simulink model "Power_Sensors"  (R2026b)
settings: Solver=VariableStepAuto
undefined symbols (not defined in the file or in its folder): DiscIntNeverNeededParam, P, Ts
libraries: eeGeneralControl x3, simulink x1
settings Model: Creator=aomar  LastModifiedBy=aomar

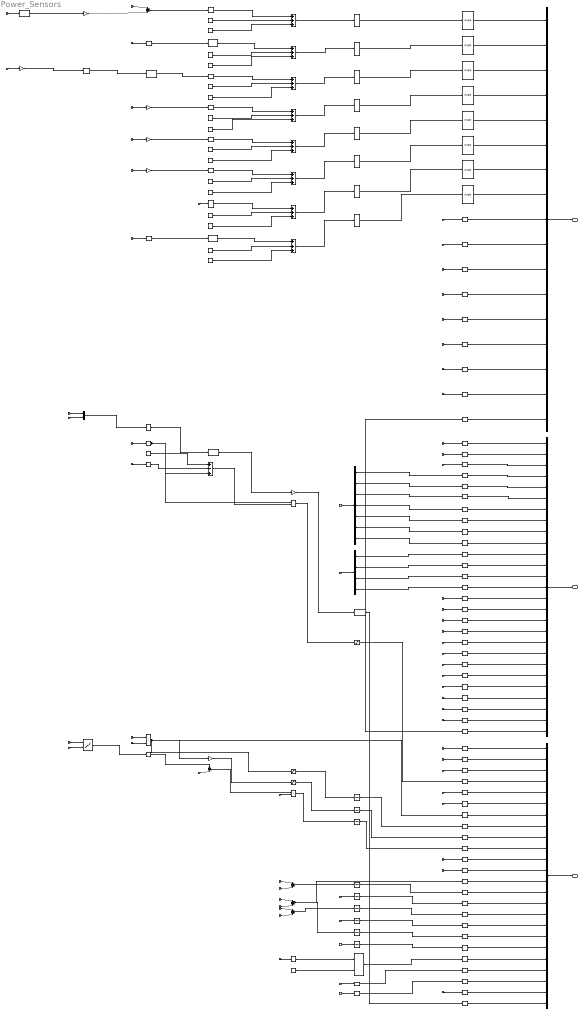
== system Power_Sensors ==
  pack_V_cell_true : Inport  PortName=pack  Element=V_cell_true
  pack_V_cell_true_2 : Inport  PortName=pack  Element=V_cell_true
  pack_T_cell_true : Inport  PortName=pack  Element=T_cell_true
  pack_T_cell_true_{2..5} (4 alike) : Inport  PortName=pack  Element=T_cell_true
  pack_SOC_true : Inport  PortName=pack  Element=SOC_true
  pack_SOC_true_2 : Inport  PortName=pack  Element=SOC_true
  pack_SOC_true_3 : Inport  PortName=pack  Element=SOC_true
  pack_SOC_true_4 : Inport  PortName=pack  Element=SOC_true
  thermal_T_air : Inport  Port=2  PortName=thermal  Element=T_air
  pdu_I_pack : Inport  Port=3  PortName=pdu  Element=I_pack
  pdu_I_pack_{2..6} (5 alike) : Inport  Port=3  PortName=pdu  Element=I_pack
  pdu_V_pack : Inport  Port=3  PortName=pdu  Element=V_pack
  pdu_V_pack_{2..5} (4 alike) : Inport  Port=3  PortName=pdu  Element=V_pack
  pdu_V_bus : Inport  Port=3  PortName=pdu  Element=V_bus
  pdu_V_bus_2 : Inport  Port=3  PortName=pdu  Element=V_bus
  pdu_V_dock : Inport  Port=3  PortName=pdu  Element=V_dock
  pdu_fuse_ok : Inport  Port=3  PortName=pdu  Element=fuse_ok
  pdu_K1_closed : Inport  Port=3  PortName=pdu  Element=K1_closed
  pdu_K1_closed_2 : Inport  Port=3  PortName=pdu  Element=K1_closed
  pdu_K1_closed_3 : Inport  Port=3  PortName=pdu  Element=K1_closed
  pdu_K2_closed : Inport  Port=3  PortName=pdu  Element=K2_closed
  pdu_K2_closed_2 : Inport  Port=3  PortName=pdu  Element=K2_closed
  pdu_K4_closed : Inport  Port=3  PortName=pdu  Element=K4_closed
  pdu_K4_closed_2 : Inport  Port=3  PortName=pdu  Element=K4_closed
  pdu_F_MAIN_ok : Inport  Port=3  PortName=pdu  Element=F_MAIN_ok
  pdu_P_trac_L : Inport  Port=3  PortName=pdu  Element=P_trac_L
  pdu_P_trac_R : Inport  Port=3  PortName=pdu  Element=P_trac_R
  pdu_P_bms : Inport  Port=3  PortName=pdu  Element=P_bms
  pdu_P_pdu_loss : Inport  Port=3  PortName=pdu  Element=P_pdu_loss
  pdu_P_chg_bus : Inport  Port=3  PortName=pdu  Element=P_chg_bus
  lv_fuse24_ok : Inport  Port=4  PortName=lv  Element=fuse24_ok
  lv_rails : Inport  Port=4  PortName=lv  Element=rails
  lv_rail_ok : Inport  Port=4  PortName=lv  Element=rail_ok
  lv_K3_closed : Inport  Port=4  PortName=lv  Element=K3_closed
  lv_P_lv : Inport  Port=4  PortName=lv  Element=P_lv
  lv_P_k3_loss : Inport  Port=4  PortName=lv  Element=P_k3_loss
  lv_P_dcdc_loss : Inport  Port=4  PortName=lv  Element=P_dcdc_loss
  lv_P_dcdc_loss_2 : Inport  Port=4  PortName=lv  Element=P_dcdc_loss
  safety_dock_present : Inport  Port=5  PortName=safety  Element=dock_present
  safety_dock_present_2 : Inport  Port=5  PortName=safety  Element=dock_present
  safety_Safety_OK : Inport  Port=5  PortName=safety  Element=Safety_OK
  safety_Safety_OK_2 : Inport  Port=5  PortName=safety  Element=Safety_OK
  safety_Safety_HV_OK : Inport  Port=5  PortName=safety  Element=Safety_HV_OK
  safety_Safety_HV_OK_2 : Inport  Port=5  PortName=safety  Element=Safety_HV_OK
  safety_key_on : Inport  Port=5  PortName=safety  Element=key_on
  safety_key_on_2 : Inport  Port=5  PortName=safety  Element=key_on
  safety_EStop_Any : Inport  Port=5  PortName=safety  Element=EStop_Any
  safety_EStop_Ch1_OK : Inport  Port=5  PortName=safety  Element=EStop_Ch1_OK
  safety_EStop_Ch2_OK : Inport  Port=5  PortName=safety  Element=EStop_Ch2_OK
  safety_Safety_Latched_Off : Inport  Port=5  PortName=safety  Element=Safety_Latched_Off
  impl_P_impl : Inport  Port=6  PortName=impl  Element=P_impl
  charger_P_grid : Inport  Port=7  PortName=charger  Element=P_grid
  env_T_amb : Inport  Port=8  PortName=env  Element=T_amb
  flt_bms_fault : Inport  Port=9  PortName=flt  Element=bms_fault
  BMS_Meas_BC : BusCreator  Inputs=17  OutDataTypeStr=Bus: Bus_BMS_Meas  NonVirtualBus=on
      settings: InheritFromInputs=off
  Fuse_Blown_u8 : DataTypeConversion  OutDataTypeStr=uint8  RndMeth=Nearest
  Fuse_ok : Mux  Inputs=2
  I_abs : Abs  SaturateOnIntegerOverflow=off
  I_peak : simulink/Math Operations/MinMax Running Resettable  Function=max  vinit=0.0
  I_peak_reset : Constant  Value=false  OutDataTypeStr=boolean  SampleTime=Ts.base
  Int_E_chg_bus : DiscreteIntegrator  gainval=1/3600  SampleTime=Ts.base  ICPrevOutput=DiscIntNeverNeededParam  ICPrevScaledInput=DiscIntNeverNeededParam
  Int_E_dcdc_loss : DiscreteIntegrator  gainval=1/3600  SampleTime=Ts.base  ICPrevOutput=DiscIntNeverNeededParam  ICPrevScaledInput=DiscIntNeverNeededParam
  Int_E_impl_dc : DiscreteIntegrator  gainval=1/3600  SampleTime=Ts.base  ICPrevOutput=DiscIntNeverNeededParam  ICPrevScaledInput=DiscIntNeverNeededParam
  Int_E_in : DiscreteIntegrator  gainval=1/3600  SampleTime=Ts.base  ICPrevOutput=DiscIntNeverNeededParam  ICPrevScaledInput=DiscIntNeverNeededParam
  Int_E_loss_batt : DiscreteIntegrator  gainval=1/3600  SampleTime=Ts.base  ICPrevOutput=DiscIntNeverNeededParam  ICPrevScaledInput=DiscIntNeverNeededParam
  Int_E_lv : DiscreteIntegrator  gainval=1/3600  SampleTime=Ts.base  ICPrevOutput=DiscIntNeverNeededParam  ICPrevScaledInput=DiscIntNeverNeededParam
  Int_E_out : DiscreteIntegrator  gainval=1/3600  SampleTime=Ts.base  ICPrevOutput=DiscIntNeverNeededParam  ICPrevScaledInput=DiscIntNeverNeededParam
  Int_E_pdu_loss : DiscreteIntegrator  gainval=1/3600  SampleTime=Ts.base  ICPrevOutput=DiscIntNeverNeededParam  ICPrevScaledInput=DiscIntNeverNeededParam
  Int_E_trac_dc : DiscreteIntegrator  gainval=1/3600  SampleTime=Ts.base  ICPrevOutput=DiscIntNeverNeededParam  ICPrevScaledInput=DiscIntNeverNeededParam
  Ipack_LPF : eeGeneralControl/Low-Pass Filter (Discrete or Continuous)  K=1  T=P.power.sensors.Ipack.tau  B=inf  A=-inf  init_option=Inherited from block input  x0=0  Ts=Ts.base
  Ipack_ZOH : ZeroOrderHold  SampleTime=Ts.afe
  Ipack_bias : Bias  Bias=P.power.sensors.Ipack.offset  SaturateOnIntegerOverflow=off
  Ipack_gain : Gain  Gain=1 + P.power.sensors.Ipack.gain_err
  Ipack_noise : RandomNumber  Mean=zeros(1,1)  Variance=P.power.sensors.Ipack.sigma^2  Seed=P.power.sensors.seed + 33  SampleTime=Ts.afe
  Ipack_offset : Constant  Value=0  SampleTime=Ts.afe
  Ipack_q : DataTypeConversion  OutDataTypeStr=single  SaturateOnIntegerOverflow=off  RndMeth=Floor
  Ipack_quant : Quantizer  QuantizationInterval=P.power.sensors.Ipack.q
  Ipack_sum : Sum  Inputs=+++
  OCV_lookup : Lookup_n-D  BreakpointsForDimension1=P.power.cell.SOC_bp  BreakpointsForDimension2=P.power.cell.T_bp  Table=P.power.cell.OCV_tab  ExtrapMethod=Clip  InternalRulePriority=Speed  RndMeth=Simplest
      settings: InputPortMap=u0,u1
  OCV_sum : Sum  Inputs=+
  P_in_pos : Saturate  UpperLimit=inf  LowerLimit=0
  P_loss_batt : Product
  P_lv_total : Sum
  P_neg : Gain  Gain=-1
  P_out_pos : Saturate  UpperLimit=inf  LowerLimit=0
  P_pack : Product
  P_pdu_total : Sum
  P_trac : Sum
  PowerStatus_BC : BusCreator  Inputs=27  OutDataTypeStr=Bus: Bus_PowerStatus  NonVirtualBus=on
      settings: InheritFromInputs=off
  PowerTruth_BC : BusCreator  Inputs=24  OutDataTypeStr=Bus: Bus_PowerTruth  NonVirtualBus=on
      settings: InheritFromInputs=off
  SOC_den : Sum  Inputs=+-+
  SOC_max : MinMax  Function=max
  SOC_min : MinMax
  SOC_pack_div : Product  Inputs=*/
  SOC_pack_sat : Saturate  UpperLimit=1  LowerLimit=0
  T_max : MinMax  Function=max
  T_min : MinMax
  Tair_NTC_lag : eeGeneralControl/Low-Pass Filter (Discrete or Continuous)  K=1  T=P.power.sensors.Tcell.tau  B=inf  A=-inf  init_option=Inherited from block input  x0=0  Ts=Ts.afe
  Tair_ZOH : ZeroOrderHold  SampleTime=Ts.afe
  Tair_noise : RandomNumber  Mean=zeros(1,1)  Variance=P.power.sensors.Tcell.sigma^2  Seed=P.power.sensors.seed + 37  SampleTime=Ts.afe
  Tair_offset : Constant  Value=0  SampleTime=Ts.afe
  Tair_q : DataTypeConversion  OutDataTypeStr=single  SaturateOnIntegerOverflow=off  RndMeth=Floor
  Tair_quant : Quantizer  QuantizationInterval=P.power.sensors.Tcell.q
  Tair_sum : Sum  Inputs=+++
  Tamb_RT : RateTransition  OutPortSampleTime=Ts.afe
  Tamb_noise : RandomNumber  Mean=zeros(1,1)  Variance=P.power.sensors.Tcell.sigma^2  Seed=P.power.sensors.seed + 38  SampleTime=Ts.afe
  Tamb_offset : Constant  Value=0  SampleTime=Ts.afe
  Tamb_q : DataTypeConversion  OutDataTypeStr=single  SaturateOnIntegerOverflow=off  RndMeth=Floor
  Tamb_quant : Quantizer  QuantizationInterval=P.power.sensors.Tcell.q
  Tamb_sum : Sum  Inputs=+++
  Tcell_NTC_lag : eeGeneralControl/Low-Pass Filter (Discrete or Continuous)  K=1  T=P.power.sensors.Tcell.tau  B=inf  A=-inf  init_option=Inherited from block input  x0=0  Ts=Ts.afe
  Tcell_ZOH : ZeroOrderHold  SampleTime=Ts.afe
  Tcell_noise : RandomNumber  Mean=zeros(P.power.pack.Ns,1)  Variance=P.power.sensors.Tcell.sigma^2  Seed=P.power.sensors.seed + (P.power.pack.Ns+1:2*P.power.pack.Ns)'  SampleTime=Ts.afe
  Tcell_offset : Constant  Value=P.power.sensors.Tcell.offset(:)  SampleTime=Ts.afe
  Tcell_q : DataTypeConversion  OutDataTypeStr=single  SaturateOnIntegerOverflow=off  RndMeth=Floor
  Tcell_quant : Quantizer  QuantizationInterval=P.power.sensors.Tcell.q
  Tcell_sum : Sum  Inputs=+++
  Vbus_ZOH : ZeroOrderHold  SampleTime=Ts.afe
  Vbus_gain : Gain  Gain=1 + P.power.sensors.Vpack.gain_err
  Vbus_noise : RandomNumber  Mean=zeros(1,1)  Variance=P.power.sensors.Vpack.sigma^2  Seed=P.power.sensors.seed + 35  SampleTime=Ts.afe
  Vbus_offset : Constant  Value=0  SampleTime=Ts.afe
  Vbus_q : DataTypeConversion  OutDataTypeStr=single  SaturateOnIntegerOverflow=off  RndMeth=Floor
  Vbus_quant : Quantizer  QuantizationInterval=P.power.sensors.Vpack.q
  Vbus_sum : Sum  Inputs=+++
  Vcell_ZOH : ZeroOrderHold  SampleTime=Ts.afe
  Vcell_fault : Sum
  Vcell_noise : RandomNumber  Mean=zeros(P.power.pack.Ns,1)  Variance=P.power.sensors.Vcell.sigma^2  Seed=P.power.sensors.seed + (1:P.power.pack.Ns)'  SampleTime=Ts.afe
  Vcell_offset : Constant  Value=P.power.sensors.Vcell.offset(:)  SampleTime=Ts.afe
  Vcell_q : DataTypeConversion  OutDataTypeStr=single  SaturateOnIntegerOverflow=off  RndMeth=Floor
  Vcell_quant : Quantizer  QuantizationInterval=P.power.sensors.Vcell.q
  Vcell_sum : Sum  Inputs=+++
  Vdock_ZOH : ZeroOrderHold  SampleTime=Ts.afe
  Vdock_gain : Gain  Gain=1 + P.power.sensors.Vpack.gain_err
  Vdock_noise : RandomNumber  Mean=zeros(1,1)  Variance=P.power.sensors.Vpack.sigma^2  Seed=P.power.sensors.seed + 36  SampleTime=Ts.afe
  Vdock_offset : Constant  Value=0  SampleTime=Ts.afe
  Vdock_q : DataTypeConversion  OutDataTypeStr=single  SaturateOnIntegerOverflow=off  RndMeth=Floor
  Vdock_quant : Quantizer  QuantizationInterval=P.power.sensors.Vpack.q
  Vdock_sum : Sum  Inputs=+++
  Vpack_ZOH : ZeroOrderHold  SampleTime=Ts.afe
  Vpack_gain : Gain  Gain=1 + P.power.sensors.Vpack.gain_err
  Vpack_noise : RandomNumber  Mean=zeros(1,1)  Variance=P.power.sensors.Vpack.sigma^2  Seed=P.power.sensors.seed + 34  SampleTime=Ts.afe
  Vpack_offset : Constant  Value=0  SampleTime=Ts.afe
  Vpack_q : DataTypeConversion  OutDataTypeStr=single  SaturateOnIntegerOverflow=off  RndMeth=Floor
  Vpack_quant : Quantizer  QuantizationInterval=P.power.sensors.Vpack.q
  Vpack_sum : Sum  Inputs=+++
  bms_fault_V : Gain  Gain=[0.5; zeros(P.power.pack.Ns-1,1)]
  bms_fault_dbl : DataTypeConversion  OutDataTypeStr=double  SaturateOnIntegerOverflow=off  RndMeth=Floor
  dV_internal : Sum  Inputs=+-
  fuse_bits_dbl : DataTypeConversion  OutDataTypeStr=double  SaturateOnIntegerOverflow=off  RndMeth=Floor
  fuse_blown_bits : Logic  Operator=NOT  AllPortsSameDT=off  OutDataTypeStr=boolean
  fuse_weights : Gain  Gain=2.^(0:6)  Multiplication=Matrix(K*u)
  meas_Dock_Present : ZeroOrderHold  SampleTime=Ts.afe
  meas_FuseMain_OK : ZeroOrderHold  SampleTime=Ts.afe
  meas_Fuse_Blown : ZeroOrderHold  SampleTime=Ts.afe
  meas_K1_fb : ZeroOrderHold  SampleTime=Ts.afe
  meas_K2_fb : ZeroOrderHold  SampleTime=Ts.afe
  meas_K4_fb : ZeroOrderHold  SampleTime=Ts.afe
  meas_Key_On : ZeroOrderHold  SampleTime=Ts.afe
  meas_Safety_HV_OK : ZeroOrderHold  SampleTime=Ts.afe
  meas_Safety_OK : ZeroOrderHold  SampleTime=Ts.afe
  one : Constant  SampleTime=Ts.base
  rail_dmx : Demux
  rails_dmx : Demux  Outputs=7
  st_Dock_Present : ZeroOrderHold  SampleTime=Ts.base
  st_EStop_Any : ZeroOrderHold  SampleTime=Ts.base
  st_EStop_Ch1_OK : ZeroOrderHold  SampleTime=Ts.base
  st_EStop_Ch2_OK : ZeroOrderHold  SampleTime=Ts.base
  st_Fuse_Blown : ZeroOrderHold  SampleTime=Ts.base
  st_I_12V_A : ZeroOrderHold  SampleTime=Ts.base
  st_I_24V_A : ZeroOrderHold  SampleTime=Ts.base
  st_I_pack_A : ZeroOrderHold  SampleTime=Ts.base
  st_K1_Closed : ZeroOrderHold  SampleTime=Ts.base
  st_K2_Closed : ZeroOrderHold  SampleTime=Ts.base
  st_K3_Closed : ZeroOrderHold  SampleTime=Ts.base
  st_K4_Closed : ZeroOrderHold  SampleTime=Ts.base
  st_Key_On : ZeroOrderHold  SampleTime=Ts.base
  st_Rail_12V_OK : ZeroOrderHold  SampleTime=Ts.base
  st_Rail_24V_OK : ZeroOrderHold  SampleTime=Ts.base
  st_Rail_3V3_OK : ZeroOrderHold  SampleTime=Ts.base
  st_Rail_5V_OK : ZeroOrderHold  SampleTime=Ts.base
  st_Safety_HV_OK : ZeroOrderHold  SampleTime=Ts.base
  st_Safety_Latched_Off : ZeroOrderHold  SampleTime=Ts.base
  st_Safety_OK : ZeroOrderHold  SampleTime=Ts.base
  st_V_12V_V : ZeroOrderHold  SampleTime=Ts.base
  st_V_24IMP_V : ZeroOrderHold  SampleTime=Ts.base
  st_V_24V_V : ZeroOrderHold  SampleTime=Ts.base
  st_V_3V3_V : ZeroOrderHold  SampleTime=Ts.base
  st_V_5V_V : ZeroOrderHold  SampleTime=Ts.base
  st_V_bus_V : ZeroOrderHold  SampleTime=Ts.base
  st_V_pack_V : ZeroOrderHold  SampleTime=Ts.base
  tr_E_chg_bus_Wh : ZeroOrderHold  SampleTime=Ts.hk
  tr_E_dcdc_loss_Wh : ZeroOrderHold  SampleTime=Ts.hk
  tr_E_impl_dc_Wh : ZeroOrderHold  SampleTime=Ts.hk
  tr_E_in_Wh : ZeroOrderHold  SampleTime=Ts.hk
  tr_E_loss_batt_Wh : ZeroOrderHold  SampleTime=Ts.hk
  tr_E_lv_Wh : ZeroOrderHold  SampleTime=Ts.hk
  tr_E_out_Wh : ZeroOrderHold  SampleTime=Ts.hk
  tr_E_pdu_loss_Wh : ZeroOrderHold  SampleTime=Ts.hk
  tr_E_trac_dc_Wh : ZeroOrderHold  SampleTime=Ts.hk
  tr_I_pack_A : ZeroOrderHold  SampleTime=Ts.hk
  tr_I_pack_peak_A : ZeroOrderHold  SampleTime=Ts.hk
  tr_P_dcdc_loss_W : ZeroOrderHold  SampleTime=Ts.hk
  tr_P_grid_W : ZeroOrderHold  SampleTime=Ts.hk
  tr_P_pack_W : ZeroOrderHold  SampleTime=Ts.hk
  tr_P_pdu_loss_W : ZeroOrderHold  SampleTime=Ts.hk
  tr_SOC_pack_true : ZeroOrderHold  SampleTime=Ts.hk
  tr_SOC_true : ZeroOrderHold  SampleTime=Ts.hk
  tr_T_cell_max_K : ZeroOrderHold  SampleTime=Ts.hk
  tr_T_cell_min_K : ZeroOrderHold  SampleTime=Ts.hk
  tr_T_cell_true : ZeroOrderHold  SampleTime=Ts.hk
  tr_V_cell_true : ZeroOrderHold  SampleTime=Ts.hk
  tr_V_term_V : ZeroOrderHold  SampleTime=Ts.hk
  tr_contactor_closed : ZeroOrderHold  SampleTime=Ts.hk
  tr_fuse_blown : ZeroOrderHold  SampleTime=Ts.hk
  bms_meas : Outport  OutDataTypeStr=Bus: Bus_BMS_Meas
  power_status : Outport  Port=2  OutDataTypeStr=Bus: Bus_PowerStatus
  power_truth : Outport  Port=3  OutDataTypeStr=Bus: Bus_PowerTruth
  wires:
  flt_bms_fault/1 -> bms_fault_dbl/1  "bms_fault"
  pdu_I_pack/1 -> Ipack_gain/1  "I_pack"
  Ipack_gain/1 -> Ipack_bias/1  "Ipack_gain"
  bms_fault_dbl/1 -> bms_fault_V/1  "bms_fault_dbl"
  pdu_fuse_ok/1 -> Fuse_ok/1  "fuse_ok"
  lv_fuse24_ok/1 -> Fuse_ok/2  "fuse24_ok"
  pack_SOC_true/1 -> OCV_lookup/1  "SOC_true"
  pack_T_cell_true_2/1 -> OCV_lookup/2  "T_cell_true"
  Fuse_ok/1 -> fuse_blown_bits/1  "fuse_ok"
  bms_fault_V/1 -> Vcell_fault/2  "dV_bms_fault"
  Ipack_bias/1 -> Ipack_LPF/1  "Ipack_bias"
  OCV_lookup/1 -> OCV_sum/1  "OCV_cell"
  pack_V_cell_true/1 -> Vcell_fault/1  "V_cell_true"
  pack_T_cell_true/1 -> Tcell_ZOH/1  "T_cell_true"
  pdu_V_pack/1 -> Vpack_gain/1  "V_pack"
  pdu_V_bus/1 -> Vbus_gain/1  "V_bus"
  pdu_V_dock/1 -> Vdock_gain/1  "V_dock"
  thermal_T_air/1 -> Tair_ZOH/1  "T_air"
  pack_SOC_true_2/1 -> SOC_min/1  "SOC_true"
  pack_SOC_true_3/1 -> SOC_max/1  "SOC_true"
  pdu_V_pack_3/1 -> P_pack/1  "V_pack"
  pdu_I_pack_3/1 -> P_pack/2  "I_pack"
  Vcell_fault/1 -> Vcell_ZOH/1  "V_cell_fault"
  Vpack_gain/1 -> Vpack_ZOH/1  "Vpack_gain"
  Vbus_gain/1 -> Vbus_ZOH/1  "Vbus_gain"
  Vdock_gain/1 -> Vdock_ZOH/1  "Vdock_gain"
  fuse_blown_bits/1 -> fuse_bits_dbl/1  "fuse_blown_bits"
  SOC_min/1 -> SOC_pack_div/1, SOC_den/3  "SOC_min"
  one/1 -> SOC_den/1  "one"
  SOC_max/1 -> SOC_den/2  "SOC_max"
  P_pack/1 -> tr_P_pack_W/1, P_out_pos/1, P_neg/1  "P_pack"
  OCV_sum/1 -> dV_internal/1  "OCV_pack"
  Tcell_ZOH/1 -> Tcell_NTC_lag/1  "Tcell_ZOH"
  Tair_ZOH/1 -> Tair_NTC_lag/1  "Tair_ZOH"
  Ipack_LPF/1 -> Ipack_ZOH/1  "Ipack_LPF"
  env_T_amb/1 -> Tamb_RT/1  "T_amb"
  pdu_V_pack_4/1 -> dV_internal/2  "V_pack"
  dV_internal/1 -> P_loss_batt/1  "dV_internal"
  Vcell_offset/1 -> Vcell_sum/2  "Vcell_offset"
  Vcell_noise/1 -> Vcell_sum/3  "Vcell_noise"
  Tcell_offset/1 -> Tcell_sum/2  "Tcell_offset"
  Tcell_noise/1 -> Tcell_sum/3  "Tcell_noise"
  Ipack_offset/1 -> Ipack_sum/2  "Ipack_offset"
  Ipack_noise/1 -> Ipack_sum/3  "Ipack_noise"
  Vpack_offset/1 -> Vpack_sum/2  "Vpack_offset"
  Vpack_noise/1 -> Vpack_sum/3  "Vpack_noise"
  Vbus_offset/1 -> Vbus_sum/2  "Vbus_offset"
  Vbus_noise/1 -> Vbus_sum/3  "Vbus_noise"
  Vdock_offset/1 -> Vdock_sum/2  "Vdock_offset"
  Vdock_noise/1 -> Vdock_sum/3  "Vdock_noise"
  Tamb_offset/1 -> Tamb_sum/2  "Tamb_offset"
  Tamb_noise/1 -> Tamb_sum/3  "Tamb_noise"
  Tair_offset/1 -> Tair_sum/2  "Tair_offset"
  Tair_noise/1 -> Tair_sum/3  "Tair_noise"
  SOC_den/1 -> SOC_pack_div/2  "SOC_den"
  P_neg/1 -> P_in_pos/1  "P_neg"
  Vcell_ZOH/1 -> Vcell_sum/1  "Vcell_ZOH"
  Ipack_ZOH/1 -> Ipack_sum/1  "Ipack_ZOH"
  Vpack_ZOH/1 -> Vpack_sum/1  "Vpack_ZOH"
  Vbus_ZOH/1 -> Vbus_sum/1  "Vbus_ZOH"
  Vdock_ZOH/1 -> Vdock_sum/1  "Vdock_ZOH"
  Tamb_RT/1 -> Tamb_sum/1  "Tamb_RT"
  Tcell_NTC_lag/1 -> Tcell_sum/1  "Tcell_NTC_lag"
  Tair_NTC_lag/1 -> Tair_sum/1  "Tair_NTC_lag"
  fuse_bits_dbl/1 -> fuse_weights/1  "fuse_bits_dbl"
  pdu_I_pack_4/1 -> P_loss_batt/2  "I_pack"
  pdu_P_trac_L/1 -> P_trac/1  "P_trac_L"
  pdu_P_trac_R/1 -> P_trac/2  "P_trac_R"
  pdu_P_pdu_loss/1 -> P_pdu_total/1  "P_pdu_loss"
  lv_P_k3_loss/1 -> P_pdu_total/2  "P_k3_loss"
  lv_P_lv/1 -> P_lv_total/1  "P_lv"
  pdu_P_bms/1 -> P_lv_total/2  "P_bms"
  pdu_I_pack_5/1 -> I_abs/1  "I_pack"
  P_trac/1 -> Int_E_trac_dc/1  "P_trac"
  P_pdu_total/1 -> Int_E_pdu_loss/1, tr_P_pdu_loss_W/1  "P_pdu_loss"
  P_lv_total/1 -> Int_E_lv/1  "P_lv"
  Vcell_sum/1 -> Vcell_quant/1  "Vcell_sum"
  Tcell_sum/1 -> Tcell_quant/1  "Tcell_sum"
  Ipack_sum/1 -> Ipack_quant/1  "Ipack_sum"
  Vpack_sum/1 -> Vpack_quant/1  "Vpack_sum"
  Vbus_sum/1 -> Vbus_quant/1  "Vbus_sum"
  Vdock_sum/1 -> Vdock_quant/1  "Vdock_sum"
  Tamb_sum/1 -> Tamb_quant/1  "Tamb_sum"
  Tair_sum/1 -> Tair_quant/1  "Tair_sum"
  fuse_weights/1 -> Fuse_Blown_u8/1  "fuse_word"
  SOC_pack_div/1 -> SOC_pack_sat/1  "SOC_pack_div"
  P_out_pos/1 -> Int_E_out/1  "P_out"
  P_in_pos/1 -> Int_E_in/1  "P_in"
  P_loss_batt/1 -> Int_E_loss_batt/1  "P_loss_batt"
  I_abs/1 -> I_peak/1  "I_abs"
  I_peak_reset/1 -> I_peak/2  "I_peak_reset"
  lv_rails/1 -> rails_dmx/1  "rails"
  lv_rail_ok/1 -> rail_dmx/1  "rail_ok"
  impl_P_impl/1 -> Int_E_impl_dc/1  "P_impl"
  lv_P_dcdc_loss/1 -> Int_E_dcdc_loss/1  "P_dcdc_loss"
  pdu_P_chg_bus/1 -> Int_E_chg_bus/1  "P_chg_bus"
  pack_T_cell_true_3/1 -> T_max/1  "T_cell_true"
  pack_T_cell_true_4/1 -> T_min/1  "T_cell_true"
  rails_dmx/1 -> st_V_24V_V/1  "V_24V"
  rails_dmx/2 -> st_I_24V_A/1  "I_24V"
  rails_dmx/3 -> st_V_24IMP_V/1  "V_24IMP"
  rails_dmx/4 -> st_V_12V_V/1  "V_12V"
  rails_dmx/5 -> st_I_12V_A/1  "I_12V"
  rails_dmx/6 -> st_V_5V_V/1  "V_5V"
  rails_dmx/7 -> st_V_3V3_V/1  "V_3V3"
  rail_dmx/1 -> st_Rail_24V_OK/1  "Rail_24V_OK"
  rail_dmx/2 -> st_Rail_12V_OK/1  "Rail_12V_OK"
  rail_dmx/3 -> st_Rail_5V_OK/1  "Rail_5V_OK"
  rail_dmx/4 -> st_Rail_3V3_OK/1  "Rail_3V3_OK"
  Vcell_quant/1 -> Vcell_q/1  "Vcell_quant"
  Tcell_quant/1 -> Tcell_q/1  "Tcell_quant"
  Ipack_quant/1 -> Ipack_q/1  "Ipack_quant"
  Vpack_quant/1 -> Vpack_q/1  "Vpack_quant"
  Vbus_quant/1 -> Vbus_q/1  "Vbus_quant"
  Vdock_quant/1 -> Vdock_q/1  "Vdock_quant"
  Tamb_quant/1 -> Tamb_q/1  "Tamb_quant"
  Tair_quant/1 -> Tair_q/1  "Tair_quant"
  SOC_pack_sat/1 -> tr_SOC_pack_true/1  "SOC_pack"
  T_max/1 -> tr_T_cell_max_K/1  "T_cell_max"
  T_min/1 -> tr_T_cell_min_K/1  "T_cell_min"
  Int_E_out/1 -> tr_E_out_Wh/1  "E_out"
  Int_E_in/1 -> tr_E_in_Wh/1  "E_in"
  Int_E_loss_batt/1 -> tr_E_loss_batt_Wh/1  "E_loss_batt"
  Int_E_trac_dc/1 -> tr_E_trac_dc_Wh/1  "E_trac_dc"
  Int_E_impl_dc/1 -> tr_E_impl_dc_Wh/1  "E_impl_dc"
  Int_E_lv/1 -> tr_E_lv_Wh/1  "E_lv"
  Int_E_dcdc_loss/1 -> tr_E_dcdc_loss_Wh/1  "E_dcdc_loss"
  Int_E_pdu_loss/1 -> tr_E_pdu_loss_Wh/1  "E_pdu_loss"
  Int_E_chg_bus/1 -> tr_E_chg_bus_Wh/1  "E_chg_bus"
  I_peak/1 -> tr_I_pack_peak_A/1  "I_pack_peak"
  Fuse_Blown_u8/1 -> tr_fuse_blown/1, meas_Fuse_Blown/1, st_Fuse_Blown/1  "Fuse_Blown"
  pdu_K1_closed/1 -> meas_K1_fb/1  "K1_closed"
  pdu_K2_closed/1 -> meas_K2_fb/1  "K2_closed"
  pdu_K4_closed/1 -> meas_K4_fb/1  "K4_closed"
  safety_dock_present/1 -> meas_Dock_Present/1  "dock_present"
  safety_Safety_OK/1 -> meas_Safety_OK/1  "Safety_OK"
  safety_Safety_HV_OK/1 -> meas_Safety_HV_OK/1  "Safety_HV_OK"
  safety_key_on/1 -> meas_Key_On/1  "key_on"
  pdu_F_MAIN_ok/1 -> meas_FuseMain_OK/1  "F_MAIN_ok"
  pdu_V_pack_2/1 -> st_V_pack_V/1  "V_pack"
  pdu_I_pack_2/1 -> st_I_pack_A/1  "I_pack"
  pdu_V_bus_2/1 -> st_V_bus_V/1  "V_bus"
  pdu_K1_closed_2/1 -> st_K1_Closed/1  "K1_closed"
  pdu_K2_closed_2/1 -> st_K2_Closed/1  "K2_closed"
  lv_K3_closed/1 -> st_K3_Closed/1  "K3_closed"
  pdu_K4_closed_2/1 -> st_K4_Closed/1  "K4_closed"
  safety_Safety_OK_2/1 -> st_Safety_OK/1  "Safety_OK"
  safety_Safety_HV_OK_2/1 -> st_Safety_HV_OK/1  "Safety_HV_OK"
  safety_EStop_Any/1 -> st_EStop_Any/1  "EStop_Any"
  safety_EStop_Ch1_OK/1 -> st_EStop_Ch1_OK/1  "EStop_Ch1_OK"
  safety_EStop_Ch2_OK/1 -> st_EStop_Ch2_OK/1  "EStop_Ch2_OK"
  safety_Safety_Latched_Off/1 -> st_Safety_Latched_Off/1  "Safety_Latched_Off"
  safety_dock_present_2/1 -> st_Dock_Present/1  "dock_present"
  safety_key_on_2/1 -> st_Key_On/1  "key_on"
  pack_SOC_true_4/1 -> tr_SOC_true/1  "SOC_true"
  pack_V_cell_true_2/1 -> tr_V_cell_true/1  "V_cell_true"
  pack_T_cell_true_5/1 -> tr_T_cell_true/1  "T_cell_true"
  pdu_V_pack_5/1 -> tr_V_term_V/1  "V_pack"
  pdu_I_pack_6/1 -> tr_I_pack_A/1  "I_pack"
  charger_P_grid/1 -> tr_P_grid_W/1  "P_grid"
  lv_P_dcdc_loss_2/1 -> tr_P_dcdc_loss_W/1  "P_dcdc_loss"
  pdu_K1_closed_3/1 -> tr_contactor_closed/1  "K1_closed"
  meas_K1_fb/1 -> BMS_Meas_BC/9  "K1_fb"
  meas_K2_fb/1 -> BMS_Meas_BC/10  "K2_fb"
  meas_K4_fb/1 -> BMS_Meas_BC/11  "K4_fb"
  meas_Dock_Present/1 -> BMS_Meas_BC/12  "Dock_Present"
  meas_Safety_OK/1 -> BMS_Meas_BC/13  "Safety_OK"
  meas_Safety_HV_OK/1 -> BMS_Meas_BC/14  "Safety_HV_OK"
  meas_Key_On/1 -> BMS_Meas_BC/15  "Key_On"
  meas_FuseMain_OK/1 -> BMS_Meas_BC/16  "FuseMain_OK"
  meas_Fuse_Blown/1 -> BMS_Meas_BC/17  "Fuse_Blown"
  st_V_pack_V/1 -> PowerStatus_BC/1  "V_pack_V"
  st_I_pack_A/1 -> PowerStatus_BC/2  "I_pack_A"
  st_V_bus_V/1 -> PowerStatus_BC/3  "V_bus_V"
  st_V_24V_V/1 -> PowerStatus_BC/4  "V_24V_V"
  st_I_24V_A/1 -> PowerStatus_BC/5  "I_24V_A"
  st_V_24IMP_V/1 -> PowerStatus_BC/6  "V_24IMP_V"
  st_V_12V_V/1 -> PowerStatus_BC/7  "V_12V_V"
  st_I_12V_A/1 -> PowerStatus_BC/8  "I_12V_A"
  st_V_5V_V/1 -> PowerStatus_BC/9  "V_5V_V"
  st_V_3V3_V/1 -> PowerStatus_BC/10  "V_3V3_V"
  st_Rail_24V_OK/1 -> PowerStatus_BC/11  "Rail_24V_OK"
  st_Rail_12V_OK/1 -> PowerStatus_BC/12  "Rail_12V_OK"
  st_Rail_5V_OK/1 -> PowerStatus_BC/13  "Rail_5V_OK"
  st_Rail_3V3_OK/1 -> PowerStatus_BC/14  "Rail_3V3_OK"
  st_K1_Closed/1 -> PowerStatus_BC/15  "K1_Closed"
  st_K2_Closed/1 -> PowerStatus_BC/16  "K2_Closed"
  st_K3_Closed/1 -> PowerStatus_BC/17  "K3_Closed"
  st_K4_Closed/1 -> PowerStatus_BC/18  "K4_Closed"
  st_Safety_OK/1 -> PowerStatus_BC/19  "Safety_OK"
  st_Safety_HV_OK/1 -> PowerStatus_BC/20  "Safety_HV_OK"
  st_EStop_Any/1 -> PowerStatus_BC/21  "EStop_Any"
  st_EStop_Ch1_OK/1 -> PowerStatus_BC/22  "EStop_Ch1_OK"
  st_EStop_Ch2_OK/1 -> PowerStatus_BC/23  "EStop_Ch2_OK"
  st_Safety_Latched_Off/1 -> PowerStatus_BC/24  "Safety_Latched_Off"
  st_Dock_Present/1 -> PowerStatus_BC/25  "Dock_Present"
  st_Key_On/1 -> PowerStatus_BC/26  "Key_On"
  st_Fuse_Blown/1 -> PowerStatus_BC/27  "Fuse_Blown"
  tr_SOC_true/1 -> PowerTruth_BC/1  "SOC_true"
  tr_V_cell_true/1 -> PowerTruth_BC/2  "V_cell_true"
  tr_T_cell_true/1 -> PowerTruth_BC/3  "T_cell_true"
  tr_SOC_pack_true/1 -> PowerTruth_BC/4  "SOC_pack_true"
  tr_V_term_V/1 -> PowerTruth_BC/5  "V_term_V"
  tr_I_pack_A/1 -> PowerTruth_BC/6  "I_pack_A"
  tr_P_pack_W/1 -> PowerTruth_BC/7  "P_pack_W"
  tr_E_out_Wh/1 -> PowerTruth_BC/8  "E_out_Wh"
  tr_E_in_Wh/1 -> PowerTruth_BC/9  "E_in_Wh"
  tr_E_loss_batt_Wh/1 -> PowerTruth_BC/10  "E_loss_batt_Wh"
  tr_P_grid_W/1 -> PowerTruth_BC/11  "P_grid_W"
  tr_P_dcdc_loss_W/1 -> PowerTruth_BC/12  "P_dcdc_loss_W"
  tr_P_pdu_loss_W/1 -> PowerTruth_BC/13  "P_pdu_loss_W"
  tr_E_trac_dc_Wh/1 -> PowerTruth_BC/14  "E_trac_dc_Wh"
  tr_E_impl_dc_Wh/1 -> PowerTruth_BC/15  "E_impl_dc_Wh"
  tr_E_lv_Wh/1 -> PowerTruth_BC/16  "E_lv_Wh"
  tr_E_dcdc_loss_Wh/1 -> PowerTruth_BC/17  "E_dcdc_loss_Wh"
  tr_E_pdu_loss_Wh/1 -> PowerTruth_BC/18  "E_pdu_loss_Wh"
  tr_E_chg_bus_Wh/1 -> PowerTruth_BC/19  "E_chg_bus_Wh"
  tr_I_pack_peak_A/1 -> PowerTruth_BC/20  "I_pack_peak_A"
  tr_T_cell_max_K/1 -> PowerTruth_BC/21  "T_cell_max_K"
  tr_T_cell_min_K/1 -> PowerTruth_BC/22  "T_cell_min_K"
  tr_contactor_closed/1 -> PowerTruth_BC/23  "contactor_closed"
  tr_fuse_blown/1 -> PowerTruth_BC/24  "fuse_blown"
  Vcell_q/1 -> BMS_Meas_BC/1  "V_cell_V"
  Tcell_q/1 -> BMS_Meas_BC/2  "T_cell_K"
  Ipack_q/1 -> BMS_Meas_BC/3  "I_pack_A"
  Vpack_q/1 -> BMS_Meas_BC/4  "V_pack_V"
  Vbus_q/1 -> BMS_Meas_BC/5  "V_bus_V"
  Vdock_q/1 -> BMS_Meas_BC/6  "V_dock_V"
  Tamb_q/1 -> BMS_Meas_BC/7  "T_amb_K"
  Tair_q/1 -> BMS_Meas_BC/8  "T_air_K"
  BMS_Meas_BC/1 -> bms_meas/1  "bms_meas"
  PowerStatus_BC/1 -> power_status/1  "power_status"
  PowerTruth_BC/1 -> power_truth/1  "power_truth"
